simulink model "large"
settings: Solver=FixedStepDiscrete  SolverMode=SingleTasking  StartTime=0  StopTime=1  FixedStep=.25

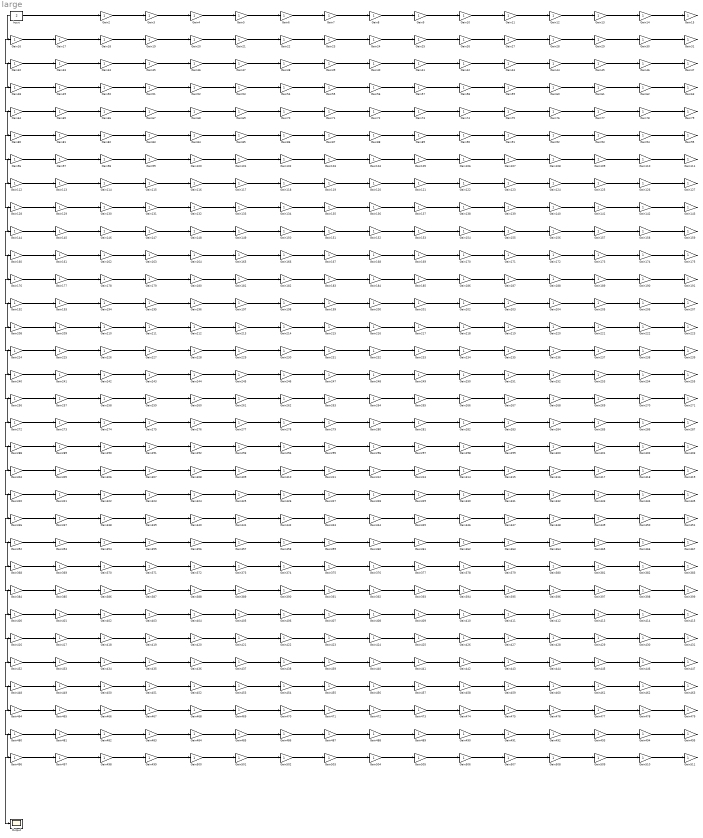
== system large ==
  Input : Constant
  Gain{2..511} (510 alike) : Gain  Gain=1  OutDataTypeStr=double
  Output : Scope
  wires:
  Input/1 -> Gain2/1
  Gain2/1 -> Gain3/1
  Gain3/1 -> Gain4/1
  Gain4/1 -> Gain5/1
  Gain5/1 -> Gain6/1
  Gain6/1 -> Gain7/1
  Gain7/1 -> Gain8/1
  Gain8/1 -> Gain9/1
  Gain9/1 -> Gain10/1
  Gain10/1 -> Gain11/1
  Gain11/1 -> Gain12/1
  Gain12/1 -> Gain13/1
  Gain13/1 -> Gain14/1
  Gain14/1 -> Gain15/1
  Gain15/1 -> Gain16/1
  Gain16/1 -> Gain17/1
  Gain17/1 -> Gain18/1
  Gain18/1 -> Gain19/1
  Gain19/1 -> Gain20/1
  Gain20/1 -> Gain21/1
  Gain21/1 -> Gain22/1
  Gain22/1 -> Gain23/1
  Gain23/1 -> Gain24/1
  Gain24/1 -> Gain25/1
  Gain25/1 -> Gain26/1
  Gain26/1 -> Gain27/1
  Gain27/1 -> Gain28/1
  Gain28/1 -> Gain29/1
  Gain29/1 -> Gain30/1
  Gain30/1 -> Gain31/1
  Gain31/1 -> Gain32/1
  Gain32/1 -> Gain33/1
  Gain33/1 -> Gain34/1
  Gain34/1 -> Gain35/1
  Gain35/1 -> Gain36/1
  Gain36/1 -> Gain37/1
  Gain37/1 -> Gain38/1
  Gain38/1 -> Gain39/1
  Gain39/1 -> Gain40/1
  Gain40/1 -> Gain41/1
  Gain41/1 -> Gain42/1
  Gain42/1 -> Gain43/1
  Gain43/1 -> Gain44/1
  Gain44/1 -> Gain45/1
  Gain45/1 -> Gain46/1
  Gain46/1 -> Gain47/1
  Gain47/1 -> Gain48/1
  Gain48/1 -> Gain49/1
  Gain49/1 -> Gain50/1
  Gain50/1 -> Gain51/1
  Gain51/1 -> Gain52/1
  Gain52/1 -> Gain53/1
  Gain53/1 -> Gain54/1
  Gain54/1 -> Gain55/1
  Gain55/1 -> Gain56/1
  Gain56/1 -> Gain57/1
  Gain57/1 -> Gain58/1
  Gain58/1 -> Gain59/1
  Gain59/1 -> Gain60/1
  Gain60/1 -> Gain61/1
  Gain61/1 -> Gain62/1
  Gain62/1 -> Gain63/1
  Gain63/1 -> Gain64/1
  Gain64/1 -> Gain65/1
  Gain65/1 -> Gain66/1
  Gain66/1 -> Gain67/1
  Gain67/1 -> Gain68/1
  Gain68/1 -> Gain69/1
  Gain69/1 -> Gain70/1
  Gain70/1 -> Gain71/1
  Gain71/1 -> Gain72/1
  Gain72/1 -> Gain73/1
  Gain73/1 -> Gain74/1
  Gain74/1 -> Gain75/1
  Gain75/1 -> Gain76/1
  Gain76/1 -> Gain77/1
  Gain77/1 -> Gain78/1
  Gain78/1 -> Gain79/1
  Gain79/1 -> Gain80/1
  Gain80/1 -> Gain81/1
  Gain81/1 -> Gain82/1
  Gain82/1 -> Gain83/1
  Gain83/1 -> Gain84/1
  Gain84/1 -> Gain85/1
  Gain85/1 -> Gain86/1
  Gain86/1 -> Gain87/1
  Gain87/1 -> Gain88/1
  Gain88/1 -> Gain89/1
  Gain89/1 -> Gain90/1
  Gain90/1 -> Gain91/1
  Gain91/1 -> Gain92/1
  Gain92/1 -> Gain93/1
  Gain93/1 -> Gain94/1
  Gain94/1 -> Gain95/1
  Gain95/1 -> Gain96/1
  Gain96/1 -> Gain97/1
  Gain97/1 -> Gain98/1
  Gain98/1 -> Gain99/1
  Gain99/1 -> Gain100/1
  Gain100/1 -> Gain101/1
  Gain101/1 -> Gain102/1
  Gain102/1 -> Gain103/1
  Gain103/1 -> Gain104/1
  Gain104/1 -> Gain105/1
  Gain105/1 -> Gain106/1
  Gain106/1 -> Gain107/1
  Gain107/1 -> Gain108/1
  Gain108/1 -> Gain109/1
  Gain109/1 -> Gain110/1
  Gain110/1 -> Gain111/1
  Gain111/1 -> Gain112/1
  Gain112/1 -> Gain113/1
  Gain113/1 -> Gain114/1
  Gain114/1 -> Gain115/1
  Gain115/1 -> Gain116/1
  Gain116/1 -> Gain117/1
  Gain117/1 -> Gain118/1
  Gain118/1 -> Gain119/1
  Gain119/1 -> Gain120/1
  Gain120/1 -> Gain121/1
  Gain121/1 -> Gain122/1
  Gain122/1 -> Gain123/1
  Gain123/1 -> Gain124/1
  Gain124/1 -> Gain125/1
  Gain125/1 -> Gain126/1
  Gain126/1 -> Gain127/1
  Gain127/1 -> Gain128/1
  Gain128/1 -> Gain129/1
  Gain129/1 -> Gain130/1
  Gain130/1 -> Gain131/1
  Gain131/1 -> Gain132/1
  Gain132/1 -> Gain133/1
  Gain133/1 -> Gain134/1
  Gain134/1 -> Gain135/1
  Gain135/1 -> Gain136/1
  Gain136/1 -> Gain137/1
  Gain137/1 -> Gain138/1
  Gain138/1 -> Gain139/1
  Gain139/1 -> Gain140/1
  Gain140/1 -> Gain141/1
  Gain141/1 -> Gain142/1
  Gain142/1 -> Gain143/1
  Gain143/1 -> Gain144/1
  Gain144/1 -> Gain145/1
  Gain145/1 -> Gain146/1
  Gain146/1 -> Gain147/1
  Gain147/1 -> Gain148/1
  Gain148/1 -> Gain149/1
  Gain149/1 -> Gain150/1
  Gain150/1 -> Gain151/1
  Gain151/1 -> Gain152/1
  Gain152/1 -> Gain153/1
  Gain153/1 -> Gain154/1
  Gain154/1 -> Gain155/1
  Gain155/1 -> Gain156/1
  Gain156/1 -> Gain157/1
  Gain157/1 -> Gain158/1
  Gain158/1 -> Gain159/1
  Gain159/1 -> Gain160/1
  Gain160/1 -> Gain161/1
  Gain161/1 -> Gain162/1
  Gain162/1 -> Gain163/1
  Gain163/1 -> Gain164/1
  Gain164/1 -> Gain165/1
  Gain165/1 -> Gain166/1
  Gain166/1 -> Gain167/1
  Gain167/1 -> Gain168/1
  Gain168/1 -> Gain169/1
  Gain169/1 -> Gain170/1
  Gain170/1 -> Gain171/1
  Gain171/1 -> Gain172/1
  Gain172/1 -> Gain173/1
  Gain173/1 -> Gain174/1
  Gain174/1 -> Gain175/1
  Gain175/1 -> Gain176/1
  Gain176/1 -> Gain177/1
  Gain177/1 -> Gain178/1
  Gain178/1 -> Gain179/1
  Gain179/1 -> Gain180/1
  Gain180/1 -> Gain181/1
  Gain181/1 -> Gain182/1
  Gain182/1 -> Gain183/1
  Gain183/1 -> Gain184/1
  Gain184/1 -> Gain185/1
  Gain185/1 -> Gain186/1
  Gain186/1 -> Gain187/1
  Gain187/1 -> Gain188/1
  Gain188/1 -> Gain189/1
  Gain189/1 -> Gain190/1
  Gain190/1 -> Gain191/1
  Gain191/1 -> Gain192/1
  Gain192/1 -> Gain193/1
  Gain193/1 -> Gain194/1
  Gain194/1 -> Gain195/1
  Gain195/1 -> Gain196/1
  Gain196/1 -> Gain197/1
  Gain197/1 -> Gain198/1
  Gain198/1 -> Gain199/1
  Gain199/1 -> Gain200/1
  Gain200/1 -> Gain201/1
  Gain201/1 -> Gain202/1
  Gain202/1 -> Gain203/1
  Gain203/1 -> Gain204/1
  Gain204/1 -> Gain205/1
  Gain205/1 -> Gain206/1
  Gain206/1 -> Gain207/1
  Gain207/1 -> Gain208/1
  Gain208/1 -> Gain209/1
  Gain209/1 -> Gain210/1
  Gain210/1 -> Gain211/1
  Gain211/1 -> Gain212/1
  Gain212/1 -> Gain213/1
  Gain213/1 -> Gain214/1
  Gain214/1 -> Gain215/1
  Gain215/1 -> Gain216/1
  Gain216/1 -> Gain217/1
  Gain217/1 -> Gain218/1
  Gain218/1 -> Gain219/1
  Gain219/1 -> Gain220/1
  Gain220/1 -> Gain221/1
  Gain221/1 -> Gain222/1
  Gain222/1 -> Gain223/1
  Gain223/1 -> Gain224/1
  Gain224/1 -> Gain225/1
  Gain225/1 -> Gain226/1
  Gain226/1 -> Gain227/1
  Gain227/1 -> Gain228/1
  Gain228/1 -> Gain229/1
  Gain229/1 -> Gain230/1
  Gain230/1 -> Gain231/1
  Gain231/1 -> Gain232/1
  Gain232/1 -> Gain233/1
  Gain233/1 -> Gain234/1
  Gain234/1 -> Gain235/1
  Gain235/1 -> Gain236/1
  Gain236/1 -> Gain237/1
  Gain237/1 -> Gain238/1
  Gain238/1 -> Gain239/1
  Gain239/1 -> Gain240/1
  Gain240/1 -> Gain241/1
  Gain241/1 -> Gain242/1
  Gain242/1 -> Gain243/1
  Gain243/1 -> Gain244/1
  Gain244/1 -> Gain245/1
  Gain245/1 -> Gain246/1
  Gain246/1 -> Gain247/1
  Gain247/1 -> Gain248/1
  Gain248/1 -> Gain249/1
  Gain249/1 -> Gain250/1
  Gain250/1 -> Gain251/1
  Gain251/1 -> Gain252/1
  Gain252/1 -> Gain253/1
  Gain253/1 -> Gain254/1
  Gain254/1 -> Gain255/1
  Gain255/1 -> Gain256/1
  Gain256/1 -> Gain257/1
  Gain257/1 -> Gain258/1
  Gain258/1 -> Gain259/1
  Gain259/1 -> Gain260/1
  Gain260/1 -> Gain261/1
  Gain261/1 -> Gain262/1
  Gain262/1 -> Gain263/1
  Gain263/1 -> Gain264/1
  Gain264/1 -> Gain265/1
  Gain265/1 -> Gain266/1
  Gain266/1 -> Gain267/1
  Gain267/1 -> Gain268/1
  Gain268/1 -> Gain269/1
  Gain269/1 -> Gain270/1
  Gain270/1 -> Gain271/1
  Gain271/1 -> Gain272/1
  Gain272/1 -> Gain273/1
  Gain273/1 -> Gain274/1
  Gain274/1 -> Gain275/1
  Gain275/1 -> Gain276/1
  Gain276/1 -> Gain277/1
  Gain277/1 -> Gain278/1
  Gain278/1 -> Gain279/1
  Gain279/1 -> Gain280/1
  Gain280/1 -> Gain281/1
  Gain281/1 -> Gain282/1
  Gain282/1 -> Gain283/1
  Gain283/1 -> Gain284/1
  Gain284/1 -> Gain285/1
  Gain285/1 -> Gain286/1
  Gain286/1 -> Gain287/1
  Gain287/1 -> Gain288/1
  Gain288/1 -> Gain289/1
  Gain289/1 -> Gain290/1
  Gain290/1 -> Gain291/1
  Gain291/1 -> Gain292/1
  Gain292/1 -> Gain293/1
  Gain293/1 -> Gain294/1
  Gain294/1 -> Gain295/1
  Gain295/1 -> Gain296/1
  Gain296/1 -> Gain297/1
  Gain297/1 -> Gain298/1
  Gain298/1 -> Gain299/1
  Gain299/1 -> Gain300/1
  Gain300/1 -> Gain301/1
  Gain301/1 -> Gain302/1
  Gain302/1 -> Gain303/1
  Gain303/1 -> Gain304/1
  Gain304/1 -> Gain305/1
  Gain305/1 -> Gain306/1
  Gain306/1 -> Gain307/1
  Gain307/1 -> Gain308/1
  Gain308/1 -> Gain309/1
  Gain309/1 -> Gain310/1
  Gain310/1 -> Gain311/1
  Gain311/1 -> Gain312/1
  Gain312/1 -> Gain313/1
  Gain313/1 -> Gain314/1
  Gain314/1 -> Gain315/1
  Gain315/1 -> Gain316/1
  Gain316/1 -> Gain317/1
  Gain317/1 -> Gain318/1
  Gain318/1 -> Gain319/1
  Gain319/1 -> Gain320/1
  Gain320/1 -> Gain321/1
  Gain321/1 -> Gain322/1
  Gain322/1 -> Gain323/1
  Gain323/1 -> Gain324/1
  Gain324/1 -> Gain325/1
  Gain325/1 -> Gain326/1
  Gain326/1 -> Gain327/1
  Gain327/1 -> Gain328/1
  Gain328/1 -> Gain329/1
  Gain329/1 -> Gain330/1
  Gain330/1 -> Gain331/1
  Gain331/1 -> Gain332/1
  Gain332/1 -> Gain333/1
  Gain333/1 -> Gain334/1
  Gain334/1 -> Gain335/1
  Gain335/1 -> Gain336/1
  Gain336/1 -> Gain337/1
  Gain337/1 -> Gain338/1
  Gain338/1 -> Gain339/1
  Gain339/1 -> Gain340/1
  Gain340/1 -> Gain341/1
  Gain341/1 -> Gain342/1
  Gain342/1 -> Gain343/1
  Gain343/1 -> Gain344/1
  Gain344/1 -> Gain345/1
  Gain345/1 -> Gain346/1
  Gain346/1 -> Gain347/1
  Gain347/1 -> Gain348/1
  Gain348/1 -> Gain349/1
  Gain349/1 -> Gain350/1
  Gain350/1 -> Gain351/1
  Gain351/1 -> Gain352/1
  Gain352/1 -> Gain353/1
  Gain353/1 -> Gain354/1
  Gain354/1 -> Gain355/1
  Gain355/1 -> Gain356/1
  Gain356/1 -> Gain357/1
  Gain357/1 -> Gain358/1
  Gain358/1 -> Gain359/1
  Gain359/1 -> Gain360/1
  Gain360/1 -> Gain361/1
  Gain361/1 -> Gain362/1
  Gain362/1 -> Gain363/1
  Gain363/1 -> Gain364/1
  Gain364/1 -> Gain365/1
  Gain365/1 -> Gain366/1
  Gain366/1 -> Gain367/1
  Gain367/1 -> Gain368/1
  Gain368/1 -> Gain369/1
  Gain369/1 -> Gain370/1
  Gain370/1 -> Gain371/1
  Gain371/1 -> Gain372/1
  Gain372/1 -> Gain373/1
  Gain373/1 -> Gain374/1
  Gain374/1 -> Gain375/1
  Gain375/1 -> Gain376/1
  Gain376/1 -> Gain377/1
  Gain377/1 -> Gain378/1
  Gain378/1 -> Gain379/1
  Gain379/1 -> Gain380/1
  Gain380/1 -> Gain381/1
  Gain381/1 -> Gain382/1
  Gain382/1 -> Gain383/1
  Gain383/1 -> Gain384/1
  Gain384/1 -> Gain385/1
  Gain385/1 -> Gain386/1
  Gain386/1 -> Gain387/1
  Gain387/1 -> Gain388/1
  Gain388/1 -> Gain389/1
  Gain389/1 -> Gain390/1
  Gain390/1 -> Gain391/1
  Gain391/1 -> Gain392/1
  Gain392/1 -> Gain393/1
  Gain393/1 -> Gain394/1
  Gain394/1 -> Gain395/1
  Gain395/1 -> Gain396/1
  Gain396/1 -> Gain397/1
  Gain397/1 -> Gain398/1
  Gain398/1 -> Gain399/1
  Gain399/1 -> Gain400/1
  Gain400/1 -> Gain401/1
  Gain401/1 -> Gain402/1
  Gain402/1 -> Gain403/1
  Gain403/1 -> Gain404/1
  Gain404/1 -> Gain405/1
  Gain405/1 -> Gain406/1
  Gain406/1 -> Gain407/1
  Gain407/1 -> Gain408/1
  Gain408/1 -> Gain409/1
  Gain409/1 -> Gain410/1
  Gain410/1 -> Gain411/1
  Gain411/1 -> Gain412/1
  Gain412/1 -> Gain413/1
  Gain413/1 -> Gain414/1
  Gain414/1 -> Gain415/1
  Gain415/1 -> Gain416/1
  Gain416/1 -> Gain417/1
  Gain417/1 -> Gain418/1
  Gain418/1 -> Gain419/1
  Gain419/1 -> Gain420/1
  Gain420/1 -> Gain421/1
  Gain421/1 -> Gain422/1
  Gain422/1 -> Gain423/1
  Gain423/1 -> Gain424/1
  Gain424/1 -> Gain425/1
  Gain425/1 -> Gain426/1
  Gain426/1 -> Gain427/1
  Gain427/1 -> Gain428/1
  Gain428/1 -> Gain429/1
  Gain429/1 -> Gain430/1
  Gain430/1 -> Gain431/1
  Gain431/1 -> Gain432/1
  Gain432/1 -> Gain433/1
  Gain433/1 -> Gain434/1
  Gain434/1 -> Gain435/1
  Gain435/1 -> Gain436/1
  Gain436/1 -> Gain437/1
  Gain437/1 -> Gain438/1
  Gain438/1 -> Gain439/1
  Gain439/1 -> Gain440/1
  Gain440/1 -> Gain441/1
  Gain441/1 -> Gain442/1
  Gain442/1 -> Gain443/1
  Gain443/1 -> Gain444/1
  Gain444/1 -> Gain445/1
  Gain445/1 -> Gain446/1
  Gain446/1 -> Gain447/1
  Gain447/1 -> Gain448/1
  Gain448/1 -> Gain449/1
  Gain449/1 -> Gain450/1
  Gain450/1 -> Gain451/1
  Gain451/1 -> Gain452/1
  Gain452/1 -> Gain453/1
  Gain453/1 -> Gain454/1
  Gain454/1 -> Gain455/1
  Gain455/1 -> Gain456/1
  Gain456/1 -> Gain457/1
  Gain457/1 -> Gain458/1
  Gain458/1 -> Gain459/1
  Gain459/1 -> Gain460/1
  Gain460/1 -> Gain461/1
  Gain461/1 -> Gain462/1
  Gain462/1 -> Gain463/1
  Gain463/1 -> Gain464/1
  Gain464/1 -> Gain465/1
  Gain465/1 -> Gain466/1
  Gain466/1 -> Gain467/1
  Gain467/1 -> Gain468/1
  Gain468/1 -> Gain469/1
  Gain469/1 -> Gain470/1
  Gain470/1 -> Gain471/1
  Gain471/1 -> Gain472/1
  Gain472/1 -> Gain473/1
  Gain473/1 -> Gain474/1
  Gain474/1 -> Gain475/1
  Gain475/1 -> Gain476/1
  Gain476/1 -> Gain477/1
  Gain477/1 -> Gain478/1
  Gain478/1 -> Gain479/1
  Gain479/1 -> Gain480/1
  Gain480/1 -> Gain481/1
  Gain481/1 -> Gain482/1
  Gain482/1 -> Gain483/1
  Gain483/1 -> Gain484/1
  Gain484/1 -> Gain485/1
  Gain485/1 -> Gain486/1
  Gain486/1 -> Gain487/1
  Gain487/1 -> Gain488/1
  Gain488/1 -> Gain489/1
  Gain489/1 -> Gain490/1
  Gain490/1 -> Gain491/1
  Gain491/1 -> Gain492/1
  Gain492/1 -> Gain493/1
  Gain493/1 -> Gain494/1
  Gain494/1 -> Gain495/1
  Gain495/1 -> Gain496/1
  Gain496/1 -> Gain497/1
  Gain497/1 -> Gain498/1
  Gain498/1 -> Gain499/1
  Gain499/1 -> Gain500/1
  Gain500/1 -> Gain501/1
  Gain501/1 -> Gain502/1
  Gain502/1 -> Gain503/1
  Gain503/1 -> Gain504/1
  Gain504/1 -> Gain505/1
  Gain505/1 -> Gain506/1
  Gain506/1 -> Gain507/1
  Gain507/1 -> Gain508/1
  Gain508/1 -> Gain509/1
  Gain509/1 -> Gain510/1
  Gain510/1 -> Gain511/1
  Gain511/1 -> Output/1
